simulink model "Residential_grid8"  (R2026a)
settings: Solver=VariableStepAuto  StopTime=365*24*3600
undefined symbols (not defined in the file): evCharge, load1, load2, load3, load4, load5, Solar, Wind
libraries: fl_lib x139, nesl_utility x68
(part 3 of 3)

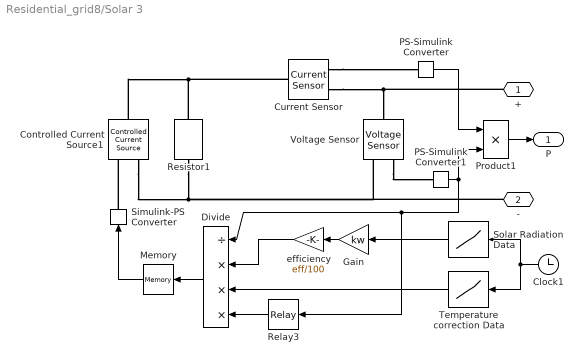
== system Residential_grid8/Solar 3 ==
  Clock1 : Clock
  Controlled Current Source1 : fl_lib/Electrical/Electrical Sources/Controlled Current Source
  Current Sensor : fl_lib/Electrical/Electrical Sensors/Current Sensor
  Divide : Product  Inputs=/***
  Gain : Gain  Gain=kw
  Memory : Memory
  PS-Simulink Converter : nesl_utility/PS-Simulink Converter  PhysicalDomain=network_engine_domain  SubClassName=ps_output  LeftPortType=input  RightPortType=output  PseudoPeriodic=off  Frequencies=[]  VectorFormat=inherit  Unit=inherit  AffineConversion=off
  PS-Simulink Converter1 : nesl_utility/PS-Simulink Converter  PhysicalDomain=network_engine_domain  SubClassName=ps_output  LeftPortType=input  RightPortType=output  PseudoPeriodic=off  Frequencies=[]  VectorFormat=inherit  Unit=inherit  AffineConversion=off
  Product1 : Product
  Relay3 : Relay  OnSwitchValue=V_stop  OffSwitchValue=V_resum  OnOutputValue=0  OffOutputValue=1
  Resistor1 : fl_lib/Electrical/Electrical Elements/Resistor  R=1e10 Ohm  i_specify=off  i_priority=None  i=0 A  i_nominal_specify=off  i_nominal_value=1  i_nominal_unit=A  v_specify=off  v_priority=None  v=0 V  v_nominal_specify=off  v_nominal_value=1  v_nominal_unit=V
  Simulink-PS Converter : nesl_utility/Simulink-PS Converter  PhysicalDomain=network_engine_domain  SubClassName=ps_input  LeftPortType=input  RightPortType=output  PseudoPeriodic=off  Frequencies=[]  NoiseDistribution=none  NoiseParameters=[]  Unit=1  AffineConversion=off  FilteringAndDerivatives=provide  SimscapeFilterOrder=1  InputFilterTimeConstant=0.001  UdotUserProvided=0
  Solar Radiation Data : Lookup_n-D  NumberOfTableDimensions=1  BreakpointsForDimension1=timestep  BeginIndexSearchUsingPreviousIndexResult=on  Table=POA  InternalRulePriority=Speed  RndMeth=Simplest
  Temperature correction Data : Lookup_n-D  NumberOfTableDimensions=1  BreakpointsForDimension1=timestep  BeginIndexSearchUsingPreviousIndexResult=on  Table=Coef  InternalRulePriority=Speed  RndMeth=Simplest
  Voltage Sensor : fl_lib/Electrical/Electrical Sensors/Voltage Sensor
  efficiency : Gain  Gain=eff/100
  + : PMIOPort  Side=Right
  - : PMIOPort  Port=2  Side=Right
  P : Outport
  wires:
  Divide/1 -> Memory/1
  Clock1/1 -> Temperature correction Data/1, Solar Radiation Data/1
  Solar Radiation Data/1 -> Gain/1
  Product1/1 -> P/1
  Gain/1 -> efficiency/1
  Memory/1 -> Simulink-PS Converter/1
  PS-Simulink Converter1/1 -> Relay3/1, Divide/1, Product1/2
  PS-Simulink Converter/1 -> Product1/1
  Temperature correction Data/1 -> Divide/3
  efficiency/1 -> Divide/2
  Relay3/1 -> Divide/4
  connections:
  Controlled Current Source1/RConn2 -- Resistor1/RConn1 -- -/RConn1 -- Voltage Sensor/RConn2
  Controlled Current Source1/LConn1 -- Current Sensor/LConn1 -- Resistor1/LConn1
  +/RConn1 -- Current Sensor/RConn2 -- Voltage Sensor/LConn1
  Current Sensor/RConn1 -- PS-Simulink Converter/LConn1
  Voltage Sensor/RConn1 -- PS-Simulink Converter1/LConn1
  Simulink-PS Converter/RConn1 -- Controlled Current Source1/RConn1

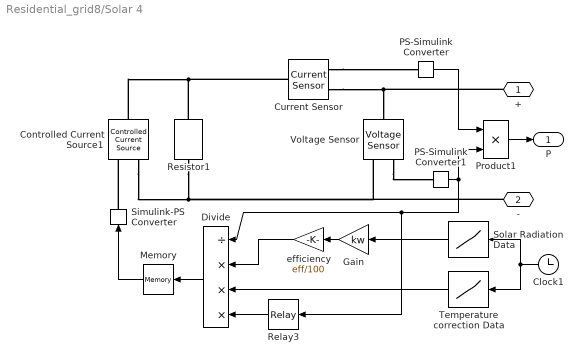
== system Residential_grid8/Solar 4 ==
  Clock1 : Clock
  Controlled Current Source1 : fl_lib/Electrical/Electrical Sources/Controlled Current Source
  Current Sensor : fl_lib/Electrical/Electrical Sensors/Current Sensor
  Divide : Product  Inputs=/***
  Gain : Gain  Gain=kw
  Memory : Memory
  PS-Simulink Converter : nesl_utility/PS-Simulink Converter  PhysicalDomain=network_engine_domain  SubClassName=ps_output  LeftPortType=input  RightPortType=output  PseudoPeriodic=off  Frequencies=[]  VectorFormat=inherit  Unit=inherit  AffineConversion=off
  PS-Simulink Converter1 : nesl_utility/PS-Simulink Converter  PhysicalDomain=network_engine_domain  SubClassName=ps_output  LeftPortType=input  RightPortType=output  PseudoPeriodic=off  Frequencies=[]  VectorFormat=inherit  Unit=inherit  AffineConversion=off
  Product1 : Product
  Relay3 : Relay  OnSwitchValue=V_stop  OffSwitchValue=V_resum  OnOutputValue=0  OffOutputValue=1
  Resistor1 : fl_lib/Electrical/Electrical Elements/Resistor  R=1e10 Ohm  i_specify=off  i_priority=None  i=0 A  i_nominal_specify=off  i_nominal_value=1  i_nominal_unit=A  v_specify=off  v_priority=None  v=0 V  v_nominal_specify=off  v_nominal_value=1  v_nominal_unit=V
  Simulink-PS Converter : nesl_utility/Simulink-PS Converter  PhysicalDomain=network_engine_domain  SubClassName=ps_input  LeftPortType=input  RightPortType=output  PseudoPeriodic=off  Frequencies=[]  NoiseDistribution=none  NoiseParameters=[]  Unit=1  AffineConversion=off  FilteringAndDerivatives=provide  SimscapeFilterOrder=1  InputFilterTimeConstant=0.001  UdotUserProvided=0
  Solar Radiation Data : Lookup_n-D  NumberOfTableDimensions=1  BreakpointsForDimension1=timestep  BeginIndexSearchUsingPreviousIndexResult=on  Table=POA  InternalRulePriority=Speed  RndMeth=Simplest
  Temperature correction Data : Lookup_n-D  NumberOfTableDimensions=1  BreakpointsForDimension1=timestep  BeginIndexSearchUsingPreviousIndexResult=on  Table=Coef  InternalRulePriority=Speed  RndMeth=Simplest
  Voltage Sensor : fl_lib/Electrical/Electrical Sensors/Voltage Sensor
  efficiency : Gain  Gain=eff/100
  + : PMIOPort  Side=Right
  - : PMIOPort  Port=2  Side=Right
  P : Outport
  wires:
  Divide/1 -> Memory/1
  Clock1/1 -> Temperature correction Data/1, Solar Radiation Data/1
  Solar Radiation Data/1 -> Gain/1
  Product1/1 -> P/1
  Gain/1 -> efficiency/1
  Memory/1 -> Simulink-PS Converter/1
  PS-Simulink Converter1/1 -> Relay3/1, Divide/1, Product1/2
  PS-Simulink Converter/1 -> Product1/1
  Temperature correction Data/1 -> Divide/3
  efficiency/1 -> Divide/2
  Relay3/1 -> Divide/4
  connections:
  Controlled Current Source1/RConn2 -- Resistor1/RConn1 -- -/RConn1 -- Voltage Sensor/RConn2
  Controlled Current Source1/LConn1 -- Current Sensor/LConn1 -- Resistor1/LConn1
  +/RConn1 -- Current Sensor/RConn2 -- Voltage Sensor/LConn1
  Current Sensor/RConn1 -- PS-Simulink Converter/LConn1
  Voltage Sensor/RConn1 -- PS-Simulink Converter1/LConn1
  Simulink-PS Converter/RConn1 -- Controlled Current Source1/RConn1

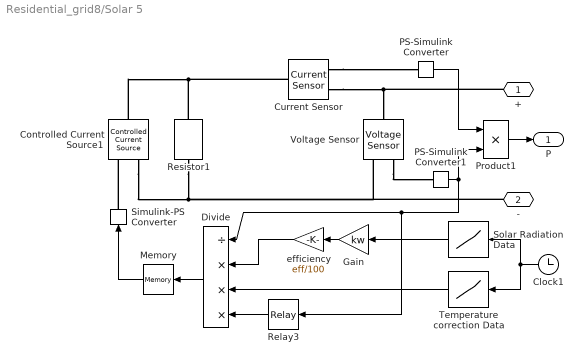
== system Residential_grid8/Solar 5 ==
  Clock1 : Clock
  Controlled Current Source1 : fl_lib/Electrical/Electrical Sources/Controlled Current Source
  Current Sensor : fl_lib/Electrical/Electrical Sensors/Current Sensor
  Divide : Product  Inputs=/***
  Gain : Gain  Gain=kw
  Memory : Memory
  PS-Simulink Converter : nesl_utility/PS-Simulink Converter  PhysicalDomain=network_engine_domain  SubClassName=ps_output  LeftPortType=input  RightPortType=output  PseudoPeriodic=off  Frequencies=[]  VectorFormat=inherit  Unit=inherit  AffineConversion=off
  PS-Simulink Converter1 : nesl_utility/PS-Simulink Converter  PhysicalDomain=network_engine_domain  SubClassName=ps_output  LeftPortType=input  RightPortType=output  PseudoPeriodic=off  Frequencies=[]  VectorFormat=inherit  Unit=inherit  AffineConversion=off
  Product1 : Product
  Relay3 : Relay  OnSwitchValue=V_stop  OffSwitchValue=V_resum  OnOutputValue=0  OffOutputValue=1
  Resistor1 : fl_lib/Electrical/Electrical Elements/Resistor  R=1e10 Ohm  i_specify=off  i_priority=None  i=0 A  i_nominal_specify=off  i_nominal_value=1  i_nominal_unit=A  v_specify=off  v_priority=None  v=0 V  v_nominal_specify=off  v_nominal_value=1  v_nominal_unit=V
  Simulink-PS Converter : nesl_utility/Simulink-PS Converter  PhysicalDomain=network_engine_domain  SubClassName=ps_input  LeftPortType=input  RightPortType=output  PseudoPeriodic=off  Frequencies=[]  NoiseDistribution=none  NoiseParameters=[]  Unit=1  AffineConversion=off  FilteringAndDerivatives=provide  SimscapeFilterOrder=1  InputFilterTimeConstant=0.001  UdotUserProvided=0
  Solar Radiation Data : Lookup_n-D  NumberOfTableDimensions=1  BreakpointsForDimension1=timestep  BeginIndexSearchUsingPreviousIndexResult=on  Table=POA  InternalRulePriority=Speed  RndMeth=Simplest
  Temperature correction Data : Lookup_n-D  NumberOfTableDimensions=1  BreakpointsForDimension1=timestep  BeginIndexSearchUsingPreviousIndexResult=on  Table=Coef  InternalRulePriority=Speed  RndMeth=Simplest
  Voltage Sensor : fl_lib/Electrical/Electrical Sensors/Voltage Sensor
  efficiency : Gain  Gain=eff/100
  + : PMIOPort  Side=Right
  - : PMIOPort  Port=2  Side=Right
  P : Outport
  wires:
  Divide/1 -> Memory/1
  Clock1/1 -> Temperature correction Data/1, Solar Radiation Data/1
  Solar Radiation Data/1 -> Gain/1
  Product1/1 -> P/1
  Gain/1 -> efficiency/1
  Memory/1 -> Simulink-PS Converter/1
  PS-Simulink Converter1/1 -> Relay3/1, Divide/1, Product1/2
  PS-Simulink Converter/1 -> Product1/1
  Temperature correction Data/1 -> Divide/3
  efficiency/1 -> Divide/2
  Relay3/1 -> Divide/4
  connections:
  Controlled Current Source1/RConn2 -- Resistor1/RConn1 -- -/RConn1 -- Voltage Sensor/RConn2
  Controlled Current Source1/LConn1 -- Current Sensor/LConn1 -- Resistor1/LConn1
  +/RConn1 -- Current Sensor/RConn2 -- Voltage Sensor/LConn1
  Current Sensor/RConn1 -- PS-Simulink Converter/LConn1
  Voltage Sensor/RConn1 -- PS-Simulink Converter1/LConn1
  Simulink-PS Converter/RConn1 -- Controlled Current Source1/RConn1

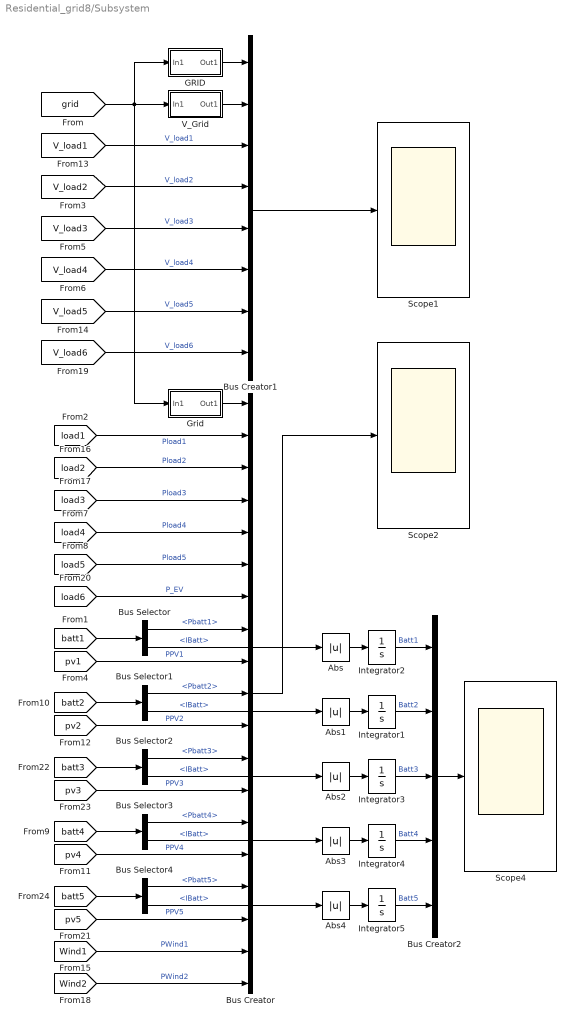
== system Residential_grid8/Subsystem ==
  Abs{,1..4} (5 alike) : Abs  SaturateOnIntegerOverflow=off
  Bus Selector : BusSelector  OutputSignals=Pbatt1,IBatt
  Bus Selector1 : BusSelector  OutputSignals=Pbatt2,IBatt
  Bus Selector2 : BusSelector  OutputSignals=Pbatt3,IBatt
  Bus Selector3 : BusSelector  OutputSignals=Pbatt4,IBatt
  Bus Selector4 : BusSelector  OutputSignals=Pbatt5,IBatt
  Bus Creator : BusCreator  Inputs=19
  Bus Creator1 : BusCreator  Inputs=8
  Bus Creator2 : BusCreator  Inputs=5
  GRID : Subsystem
  Grid : Subsystem
  Integrator{1..5} (5 alike) : Integrator  InitialCondition=1  LimitOutput=on  LowerSaturationLimit=0
  Scope1 : Scope
      settings: TimeSpan=24*365*3600  ActiveDisplayYMinimum=355  ActiveDisplayYMaximum=405  YLabel=Voltage (V)  DataLoggingDecimation=60  DataLoggingVariableName=Scope1_Data
  Scope2 : Scope
      settings: TimeSpan=24*365*3600  ActiveDisplayYMinimum=-12266.517881119289  ActiveDisplayYMaximum=11781.22849691175  YLabel=Power (W)  DataLoggingDecimation=60
  Scope4 : Scope
      settings: TimeSpan=24*365*3600  ActiveDisplayYMinimum=0  ActiveDisplayYMaximum=7.0E+7  YLabel=Accumulated Charge/Discharge Current (A Sec)  DataLoggingVariableName=ScopeData3
  V_Grid : Subsystem
  wires:
  GRID/1(Out1) -> Bus Creator1/1
  [grid] -> V_Grid/1(In1), GRID/1(In1), Grid/1(In1)
  V_Grid/1(Out1) -> Bus Creator1/2
  Grid/1(Out1) -> Bus Creator/1
  Bus Creator/1 -> Scope2/1
  [pv2] -> Bus Creator/11  "PPV2"
  [pv3] -> Bus Creator/13  "PPV3"
  [pv1] -> Bus Creator/9  "PPV1"
  [load1] -> Bus Creator/2  "Pload1"
  [load2] -> Bus Creator/3  "Pload2"
  [load3] -> Bus Creator/4  "Pload3"
  [batt1] -> Bus Selector/1
  Bus Selector/1 -> Bus Creator/8  "<Pbatt1>"
  [batt2] -> Bus Selector1/1
  Bus Selector1/1 -> Bus Creator/10  "<Pbatt2>"
  [batt3] -> Bus Selector2/1
  Bus Selector2/1 -> Bus Creator/12  "<Pbatt3>"
  [V_load2] -> Bus Creator1/4  "V_load2"
  [V_load3] -> Bus Creator1/5  "V_load3"
  [V_load4] -> Bus Creator1/6  "V_load4"
  [load4] -> Bus Creator/5  "Pload4"
  [pv4] -> Bus Creator/15  "PPV4"
  [batt4] -> Bus Selector3/1
  Bus Selector3/1 -> Bus Creator/14  "<Pbatt4>"
  [load5] -> Bus Creator/6  "Pload5"
  Bus Creator1/1 -> Scope1/1
  [V_load1] -> Bus Creator1/3  "V_load1"
  Abs1/1 -> Integrator1/1
  Abs/1 -> Integrator2/1
  Integrator1/1 -> Bus Creator2/2  "Batt2"
  Integrator3/1 -> Bus Creator2/3  "Batt3"
  Integrator4/1 -> Bus Creator2/4  "Batt4"
  Abs3/1 -> Integrator4/1
  Abs2/1 -> Integrator3/1
  Integrator2/1 -> Bus Creator2/1  "Batt1"
  Bus Creator2/1 -> Scope4/1
  Bus Selector/2 -> Abs/1  "<IBatt>"
  Bus Selector1/2 -> Abs1/1  "<IBatt>"
  Bus Selector2/2 -> Abs2/1  "<IBatt>"
  Bus Selector3/2 -> Abs3/1  "<IBatt>"
  [V_load5] -> Bus Creator1/7  "V_load5"
  [Wind1] -> Bus Creator/18  "PWind1"
  [Wind2] -> Bus Creator/19  "PWind2"
  [V_load6] -> Bus Creator1/8  "V_load6"
  [load6] -> Bus Creator/7  "P_EV"
  [pv5] -> Bus Creator/17  "PPV5"
  [batt5] -> Bus Selector4/1
  Bus Selector4/1 -> Bus Creator/16  "<Pbatt5>"
  Integrator5/1 -> Bus Creator2/5  "Batt5"
  Abs4/1 -> Integrator5/1
  Bus Selector4/2 -> Abs4/1  "<IBatt>"

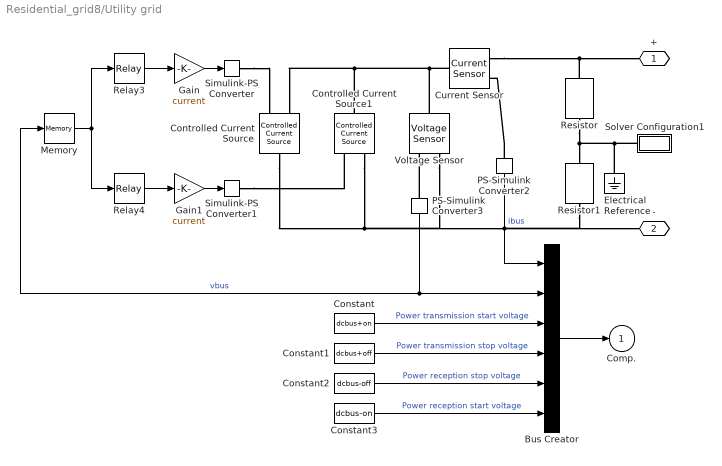
== system Residential_grid8/Utility grid ==
  Bus Creator : BusCreator  Inputs=6
  Constant : Constant  Value=dcbus+on
  Constant1 : Constant  Value=dcbus+off
  Constant2 : Constant  Value=dcbus-off
  Constant3 : Constant  Value=dcbus-on
  Controlled Current Source : fl_lib/Electrical/Electrical Sources/Controlled Current Source
  Controlled Current Source1 : fl_lib/Electrical/Electrical Sources/Controlled Current Source
  Current Sensor : fl_lib/Electrical/Electrical Sensors/Current Sensor
  Electrical Reference : fl_lib/Electrical/Electrical Elements/Electrical Reference
  Gain : Gain  Gain=current
  Gain1 : Gain  Gain=current
  Memory : Memory
  PS-Simulink Converter2 : nesl_utility/PS-Simulink Converter  PhysicalDomain=network_engine_domain  SubClassName=ps_output  LeftPortType=input  RightPortType=output  PseudoPeriodic=off  Frequencies=[]  VectorFormat=inherit  Unit=inherit  AffineConversion=off
  PS-Simulink Converter3 : nesl_utility/PS-Simulink Converter  PhysicalDomain=network_engine_domain  SubClassName=ps_output  LeftPortType=input  RightPortType=output  PseudoPeriodic=off  Frequencies=[]  VectorFormat=inherit  Unit=inherit  AffineConversion=off
  Relay3 : Relay  OnSwitchValue=dcbus+on  OffSwitchValue=dcbus+off
  Relay4 : Relay  OnSwitchValue=dcbus-off  OffSwitchValue=dcbus-on  OnOutputValue=0  OffOutputValue=1
  Resistor : fl_lib/Electrical/Electrical Elements/Resistor  R=1E6 Ohm  i_specify=off  i_priority=None  i=0 A  i_nominal_specify=off  i_nominal_value=1  i_nominal_unit=A  v_specify=off  v_priority=None  v=0 V  v_nominal_specify=off  v_nominal_value=1  v_nominal_unit=V
  Resistor1 : fl_lib/Electrical/Electrical Elements/Resistor  R=1E6 Ohm  i_specify=off  i_priority=None  i=0 A  i_nominal_specify=off  i_nominal_value=1  i_nominal_unit=A  v_specify=off  v_priority=None  v=0 V  v_nominal_specify=off  v_nominal_value=1  v_nominal_unit=V
  Simulink-PS Converter : nesl_utility/Simulink-PS Converter  PhysicalDomain=network_engine_domain  SubClassName=ps_input  LeftPortType=input  RightPortType=output  PseudoPeriodic=off  Frequencies=[]  NoiseDistribution=none  NoiseParameters=[]  Unit=1  AffineConversion=off  FilteringAndDerivatives=provide  SimscapeFilterOrder=1  InputFilterTimeConstant=0.001  UdotUserProvided=0
  Simulink-PS Converter1 : nesl_utility/Simulink-PS Converter  PhysicalDomain=network_engine_domain  SubClassName=ps_input  LeftPortType=input  RightPortType=output  PseudoPeriodic=off  Frequencies=[]  NoiseDistribution=none  NoiseParameters=[]  Unit=1  AffineConversion=off  FilteringAndDerivatives=provide  SimscapeFilterOrder=1  InputFilterTimeConstant=0.001  UdotUserProvided=0
  Solver Configuration1 : Subsystem  Priority=1  mask{TimeDomain=Continuous, UseLocalSolver=on, LocalSolverSampleTime=10, LocalSolverChoice=NE_BACKWARD_EULER_ADVANCER, DoFixedCost=on, MaxNonlinIter=4}
      settings: OpenFcn=elec.conv.unmask(gcb);
      mask TypeOptions TimeDomain: Continuous | Discrete | Phasor
      mask TypeOptions UseLocalSolver:
      | Solver
      | Configuration/UseLocalSolver
      mask TypeOptions LocalSolverSampleTime:
      | Solver
      | Configuration/LocalSolverSampleTime
      mask TypeOptions LocalSolverChoice:
      | Solver
      | Configuration/LocalSolverChoice
      mask TypeOptions DoFixedCost:
      | Solver
      | Configuration/DoFixedCost
      mask TypeOptions MaxNonlinIter:
      | Solver
      | Configuration/MaxNonlinIter
  Voltage Sensor : fl_lib/Electrical/Electrical Sensors/Voltage Sensor
  + : PMIOPort  Side=Right  ConnectionType=Connection: foundation.electrical.electrical
  - : PMIOPort  Port=2  Side=Right  ConnectionType=Connection: foundation.electrical.electrical
  Comp. : Outport
  wires:
  Memory/1 -> Relay4/1, Relay3/1
  Relay3/1 -> Gain/1
  Gain/1 -> Simulink-PS Converter/1
  Relay4/1 -> Gain1/1
  Gain1/1 -> Simulink-PS Converter1/1
  Constant1/1 -> Bus Creator/4  "Power transmission stop voltage"
  Constant/1 -> Bus Creator/3  "Power transmission start voltage"
  Constant2/1 -> Bus Creator/5  "Power reception stop voltage"
  Constant3/1 -> Bus Creator/6  "Power reception start voltage"
  Bus Creator/1 -> Comp./1
  PS-Simulink Converter3/1 -> Bus Creator/2, Memory/1  "vbus"
  PS-Simulink Converter2/1 -> Bus Creator/1  "ibus"
  connections:
  Simulink-PS Converter/RConn1 -- Controlled Current Source/RConn1
  Current Sensor/LConn1 -- Voltage Sensor/LConn1 -- Controlled Current Source1/LConn1 -- Controlled Current Source/RConn2
  Controlled Current Source/LConn1 -- Controlled Current Source1/RConn2 -- Voltage Sensor/RConn2 -- Resistor1/RConn1 -- -/RConn1
  Simulink-PS Converter1/RConn1 -- Controlled Current Source1/RConn1
  Current Sensor/RConn2 -- Resistor/LConn1 -- +/RConn1
  Electrical Reference/LConn1 -- Solver Configuration1/RConn1 -- Resistor/RConn1 -- Resistor1/LConn1
  PS-Simulink Converter2/LConn1 -- Current Sensor/RConn1
  PS-Simulink Converter3/LConn1 -- Voltage Sensor/RConn1

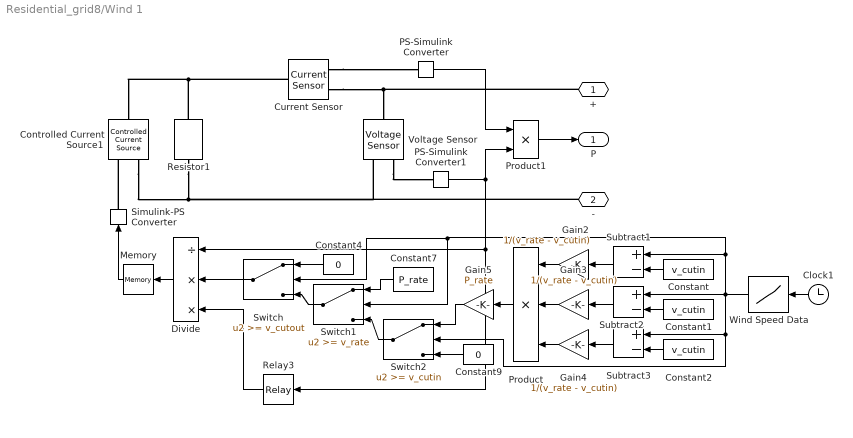
== system Residential_grid8/Wind 1 ==
  Clock1 : Clock
  Constant : Constant  Value=v_cutin
  Constant1 : Constant  Value=v_cutin
  Constant2 : Constant  Value=v_cutin
  Constant4 : Constant  Value=0
  Constant7 : Constant  Value=P_rate
  Constant9 : Constant  Value=0
  Controlled Current Source1 : fl_lib/Electrical/Electrical Sources/Controlled Current Source
  Current Sensor : fl_lib/Electrical/Electrical Sensors/Current Sensor
  Divide : Product  Inputs=/**
  Gain2 : Gain  Gain=1/(v_rate - v_cutin)
  Gain3 : Gain  Gain=1/(v_rate - v_cutin)
  Gain4 : Gain  Gain=1/(v_rate - v_cutin)
  Gain5 : Gain  Gain=P_rate
  Memory : Memory
  PS-Simulink Converter : nesl_utility/PS-Simulink Converter  PhysicalDomain=network_engine_domain  SubClassName=ps_output  LeftPortType=input  RightPortType=output  PseudoPeriodic=off  Frequencies=[]  VectorFormat=inherit  Unit=inherit  AffineConversion=off
  PS-Simulink Converter1 : nesl_utility/PS-Simulink Converter  PhysicalDomain=network_engine_domain  SubClassName=ps_output  LeftPortType=input  RightPortType=output  PseudoPeriodic=off  Frequencies=[]  VectorFormat=inherit  Unit=inherit  AffineConversion=off
  Product : Product  Inputs=3
  Product1 : Product
  Relay3 : Relay  OnSwitchValue=V_stop  OffSwitchValue=V_resum  OnOutputValue=0  OffOutputValue=1
  Resistor1 : fl_lib/Electrical/Electrical Elements/Resistor  R=1e10 Ohm  i_specify=off  i_priority=None  i=0 A  i_nominal_specify=off  i_nominal_value=1  i_nominal_unit=A  v_specify=off  v_priority=None  v=0 V  v_nominal_specify=off  v_nominal_value=1  v_nominal_unit=V
  Simulink-PS Converter : nesl_utility/Simulink-PS Converter  PhysicalDomain=network_engine_domain  SubClassName=ps_input  LeftPortType=input  RightPortType=output  PseudoPeriodic=off  Frequencies=[]  NoiseDistribution=none  NoiseParameters=[]  Unit=1  AffineConversion=off  FilteringAndDerivatives=provide  SimscapeFilterOrder=1  InputFilterTimeConstant=0.001  UdotUserProvided=0
  Subtract1 : Sum  Inputs=+-
  Subtract2 : Sum  Inputs=+-
  Subtract3 : Sum  Inputs=+-
  Switch : Switch  Threshold=v_cutout  SaturateOnIntegerOverflow=off  InputSameDT=off
  Switch1 : Switch  Threshold=v_rate  SaturateOnIntegerOverflow=off  InputSameDT=off
  Switch2 : Switch  Threshold=v_cutin  SaturateOnIntegerOverflow=off  InputSameDT=off
  Voltage Sensor : fl_lib/Electrical/Electrical Sensors/Voltage Sensor
  Wind Speed Data : Lookup_n-D  NumberOfTableDimensions=1  BreakpointsForDimension1=timestep  BeginIndexSearchUsingPreviousIndexResult=on  Table=Wind  InternalRulePriority=Speed  RndMeth=Simplest
  + : PMIOPort  Side=Right
  - : PMIOPort  Port=2  Side=Right
  P : Outport
  wires:
  Divide/1 -> Memory/1
  Clock1/1 -> Wind Speed Data/1
  Product1/1 -> P/1
  Memory/1 -> Simulink-PS Converter/1
  PS-Simulink Converter1/1 -> Divide/1, Relay3/1, Product1/2
  Gain2/1 -> Product/1
  Gain3/1 -> Product/2
  Gain4/1 -> Product/3
  Subtract1/1 -> Gain2/1
  Constant/1 -> Subtract1/2
  Constant1/1 -> Subtract2/2
  Subtract2/1 -> Gain3/1
  Subtract3/1 -> Gain4/1
  Constant2/1 -> Subtract3/2
  Product/1 -> Gain5/1
  Wind Speed Data/1 -> Subtract3/1, Switch2/2, Subtract1/1, Switch/2, Switch1/2, Subtract2/1
  Constant4/1 -> Switch/1
  Constant7/1 -> Switch1/1
  Switch1/1 -> Switch/3
  Switch2/1 -> Switch1/3
  Gain5/1 -> Switch2/1
  Constant9/1 -> Switch2/3
  PS-Simulink Converter/1 -> Product1/1
  Switch/1 -> Divide/2
  Relay3/1 -> Divide/3
  connections:
  Controlled Current Source1/RConn2 -- Resistor1/RConn1 -- -/RConn1 -- Voltage Sensor/RConn2
  Resistor1/LConn1 -- Current Sensor/LConn1 -- Controlled Current Source1/LConn1
  +/RConn1 -- Current Sensor/RConn2 -- Voltage Sensor/LConn1
  Current Sensor/RConn1 -- PS-Simulink Converter/LConn1
  Voltage Sensor/RConn1 -- PS-Simulink Converter1/LConn1
  Simulink-PS Converter/RConn1 -- Controlled Current Source1/RConn1

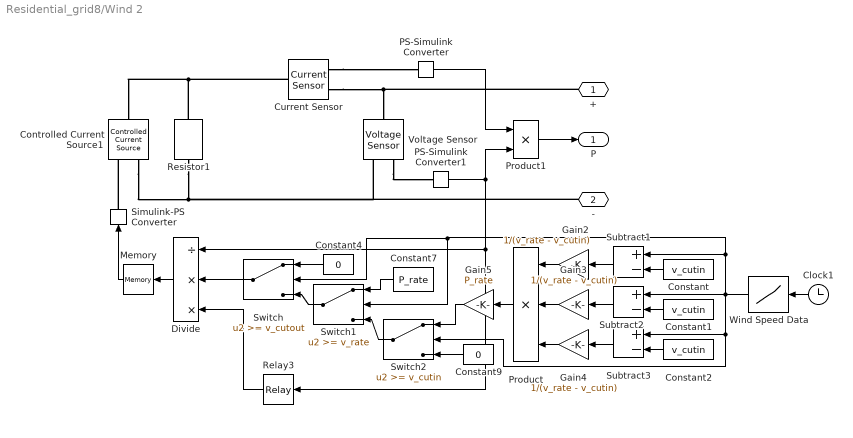
== system Residential_grid8/Wind 2 ==
  Clock1 : Clock
  Constant : Constant  Value=v_cutin
  Constant1 : Constant  Value=v_cutin
  Constant2 : Constant  Value=v_cutin
  Constant4 : Constant  Value=0
  Constant7 : Constant  Value=P_rate
  Constant9 : Constant  Value=0
  Controlled Current Source1 : fl_lib/Electrical/Electrical Sources/Controlled Current Source
  Current Sensor : fl_lib/Electrical/Electrical Sensors/Current Sensor
  Divide : Product  Inputs=/**
  Gain2 : Gain  Gain=1/(v_rate - v_cutin)
  Gain3 : Gain  Gain=1/(v_rate - v_cutin)
  Gain4 : Gain  Gain=1/(v_rate - v_cutin)
  Gain5 : Gain  Gain=P_rate
  Memory : Memory
  PS-Simulink Converter : nesl_utility/PS-Simulink Converter  PhysicalDomain=network_engine_domain  SubClassName=ps_output  LeftPortType=input  RightPortType=output  PseudoPeriodic=off  Frequencies=[]  VectorFormat=inherit  Unit=inherit  AffineConversion=off
  PS-Simulink Converter1 : nesl_utility/PS-Simulink Converter  PhysicalDomain=network_engine_domain  SubClassName=ps_output  LeftPortType=input  RightPortType=output  PseudoPeriodic=off  Frequencies=[]  VectorFormat=inherit  Unit=inherit  AffineConversion=off
  Product : Product  Inputs=3
  Product1 : Product
  Relay3 : Relay  OnSwitchValue=V_stop  OffSwitchValue=V_resum  OnOutputValue=0  OffOutputValue=1
  Resistor1 : fl_lib/Electrical/Electrical Elements/Resistor  R=1e10 Ohm  i_specify=off  i_priority=None  i=0 A  i_nominal_specify=off  i_nominal_value=1  i_nominal_unit=A  v_specify=off  v_priority=None  v=0 V  v_nominal_specify=off  v_nominal_value=1  v_nominal_unit=V
  Simulink-PS Converter : nesl_utility/Simulink-PS Converter  PhysicalDomain=network_engine_domain  SubClassName=ps_input  LeftPortType=input  RightPortType=output  PseudoPeriodic=off  Frequencies=[]  NoiseDistribution=none  NoiseParameters=[]  Unit=1  AffineConversion=off  FilteringAndDerivatives=provide  SimscapeFilterOrder=1  InputFilterTimeConstant=0.001  UdotUserProvided=0
  Subtract1 : Sum  Inputs=+-
  Subtract2 : Sum  Inputs=+-
  Subtract3 : Sum  Inputs=+-
  Switch : Switch  Threshold=v_cutout  SaturateOnIntegerOverflow=off  InputSameDT=off
  Switch1 : Switch  Threshold=v_rate  SaturateOnIntegerOverflow=off  InputSameDT=off
  Switch2 : Switch  Threshold=v_cutin  SaturateOnIntegerOverflow=off  InputSameDT=off
  Voltage Sensor : fl_lib/Electrical/Electrical Sensors/Voltage Sensor
  Wind Speed Data : Lookup_n-D  NumberOfTableDimensions=1  BreakpointsForDimension1=timestep  BeginIndexSearchUsingPreviousIndexResult=on  Table=Wind  InternalRulePriority=Speed  RndMeth=Simplest
  + : PMIOPort  Side=Right
  - : PMIOPort  Port=2  Side=Right
  P : Outport
  wires:
  Divide/1 -> Memory/1
  Clock1/1 -> Wind Speed Data/1
  Product1/1 -> P/1
  Memory/1 -> Simulink-PS Converter/1
  PS-Simulink Converter1/1 -> Divide/1, Relay3/1, Product1/2
  Gain2/1 -> Product/1
  Gain3/1 -> Product/2
  Gain4/1 -> Product/3
  Subtract1/1 -> Gain2/1
  Constant/1 -> Subtract1/2
  Constant1/1 -> Subtract2/2
  Subtract2/1 -> Gain3/1
  Subtract3/1 -> Gain4/1
  Constant2/1 -> Subtract3/2
  Product/1 -> Gain5/1
  Wind Speed Data/1 -> Subtract3/1, Switch2/2, Subtract1/1, Switch/2, Switch1/2, Subtract2/1
  Constant4/1 -> Switch/1
  Constant7/1 -> Switch1/1
  Switch1/1 -> Switch/3
  Switch2/1 -> Switch1/3
  Gain5/1 -> Switch2/1
  Constant9/1 -> Switch2/3
  PS-Simulink Converter/1 -> Product1/1
  Switch/1 -> Divide/2
  Relay3/1 -> Divide/3
  connections:
  Controlled Current Source1/RConn2 -- Resistor1/RConn1 -- -/RConn1 -- Voltage Sensor/RConn2
  Resistor1/LConn1 -- Current Sensor/LConn1 -- Controlled Current Source1/LConn1
  +/RConn1 -- Current Sensor/RConn2 -- Voltage Sensor/LConn1
  Current Sensor/RConn1 -- PS-Simulink Converter/LConn1
  Voltage Sensor/RConn1 -- PS-Simulink Converter1/LConn1
  Simulink-PS Converter/RConn1 -- Controlled Current Source1/RConn1

== system Residential_grid8/Subsystem/GRID ==
  In1 : Inport
  Bus Selector1 : BusSelector  OutputSignals=Power reception start voltage,Power reception stop voltage,Power transmission stop voltage,Power transmission start voltage
  Bus Creator : BusCreator  Inputs=4
  Out1 : Outport
  wires:
  In1/1 -> Bus Selector1/1
  Bus Creator/1 -> Out1/1
  Bus Selector1/1 -> Bus Creator/1  "<Power reception start voltage>"
  Bus Selector1/2 -> Bus Creator/2  "<Power reception stop voltage>"
  Bus Selector1/3 -> Bus Creator/3  "<Power transmission stop voltage>"
  Bus Selector1/4 -> Bus Creator/4  "<Power transmission start voltage>"

== system Residential_grid8/Subsystem/Grid ==
  In1 : Inport
  Bus Selector : BusSelector  OutputSignals=vbus,ibus
  Product1 : Product
  Out1 : Outport
  wires:
  In1/1 -> Bus Selector/1
  Bus Selector/1 -> Product1/1  "<vbus>"
  Bus Selector/2 -> Product1/2  "<ibus>"
  Product1/1 -> Out1/1  "BUS 1"

== system Residential_grid8/Subsystem/V_Grid ==
  In1 : Inport
  Bus Selector1 : BusSelector  OutputSignals=vbus
  Out1 : Outport
  wires:
  In1/1 -> Bus Selector1/1
  Bus Selector1/1 -> Out1/1  "<vbus>"

== system Residential_grid8/Utility grid/Solver Configuration1 ==
  Solver Configuration : nesl_utility/Solver Configuration  PhysicalDomain=network_engine_domain  SubClassName=solver  LeftPortType=input  RightPortType=generic  Tones=[]  Harmonics=[]  SimulateNoise=off  Profile=off  UseLocalSampling=off  EnableSwitchedLinearOptims=on  FrequencyDomain=off  UseCCode=off  RelTol=0.001  AbsTol=1e-06  MinStep=1e-09  ToWorkspace=off  RevertToSquareIcSolve=off  NumHomotopyIterations=100  PhasorMode=off  PhasorModeNumHarmonics=1  ConsistencySolver=NEWTON_FTOL  CanonicalOrdering=UNORDERED  OptimizeIntermediates=UNOPTIMIZED  IndexReductionMethod=DerivativeReplacement  DoDC=off  ResidualTolerance=1e-09  ConsistencyTolSource=GLOBAL  ConsistencyAbsTol=0.001  ConsistencyRelTol=0.001  ConsistencyTolFactor=0.001  UseLocalSolver=on  LocalSolverChoice=NE_BACKWARD_EULER_ADVANCER  ResolveIndetEquations=on  FunctionEvalNumThread=1  LocalSolverSampleTime=LocalSolverSampleTime  DoFixedCost=on  MaxNonlinIter=MaxNonlinIter  MaxModeIter=2  ComputeImpulses=off  ImpulseIterations=1  LinearAlgebra=Sparse  LinearAlgebraNumThread=0  EquationFormulation=NE_TIME_EF  DelaysMemoryBudget=1024  AutomaticFiltering=on  FilteringTimeConstant=0.001  PartitionStorageMethod=AS_NEEDED  PartitionMemoryBudget=1024  PartitionMethod=FAST  MultibodyUseLocalSolver=off  MultibodyLocalSolverChoice=ODE1  MultibodyLocalSolverSampleTime=0.001
  f(x)=0 : PMIOPort  Side=Right
  connections:
  f(x)=0/RConn1 -- Solver Configuration/RConn1
